simulink model "mars_rover_test_harness_chassis"  (R2025a)
settings: Solver=ode23t  StartTime=0.0  StopTime=30  FixedStep=1e-10  MaxStep=1e-1  RelTol=1e-3  AbsTol=1e-3  EnableMultiTasking=on
undefined symbols (not defined in the file): arm_q0, Control, L1, L2, L3, LS1, LS3, R1, R2, R3, Rover, RS1, RS3, X, Y, Z
libraries: sm_lib x119, nesl_utility x99, fl_lib x85, sdl_lib x20, ee_lib x10, mars_rover_lib x8, simulink x5, slpidlib x3, batteryecm_lib x2
(part 7 of 8)

== system mars_rover_test_harness_chassis/Rover/Chassis/Powertrain/Ideal/Power ==
  i : Inport
  Ambient Temperature : fl_lib/Thermal/Thermal Sources/Temperature Source  temperature=273+25 K
  Battery : batteryecm_lib/Battery  Vnom=14 V  prm_dir=1  R1_dis=2 Ohm  R1_ch=2 Ohm  R1=2e-3 Ohm  prm_AH=2  AH=100 A*hr  V1=11.5 V  AH1=100/2 A*hr  prm_R2=1  R2=2000 Ohm  Tmeas=298.15 K  charge_measurement_port=simscape.enum.battery.enable.yes  prm_dyn=1  Rp1=0.005 Ohm  tau1=30 s  Rp2=0.005 Ohm  tau2=30 s  Rp3=0.005 Ohm  tau3=30 s  Rp4=0.005 Ohm  tau4=30 s  Rp5=0.005 Ohm  tau5=30 s  prm_fade=1  N_fade=100  AH_fade=45 A*hr  R1_fade=2.02 Ohm  R1_ch_fade=2.02 Ohm  V1_fade=10.35 V  prm_age=1  prm_age_OCV=1  OCV_age=0.9  SOC_age=60  Tmeas_age=298.15 K  delta_time_age_vec=[0] d  temperature_age_vec=[273] K  OCV_scaling_age=2.2134e6  OCV_offset_age=1.632e6  temp_exp_age=0.515833569 V  t_exp_age=0.75  Vnom_T2=12 V  R1_T2=2e-2 Ohm  R1_T2_dis=2.2 Ohm  R1_T2_ch=2.2 Ohm  V1_T2=11.4 V  R2_T2=2200 Ohm  Rp1_T2=0.005 Ohm  tau1_T2=30 s  Rp2_T2=0.005 Ohm  tau2_T2=30 s  Rp3_T2=0.005 Ohm  tau3_T2=30 s  Rp4_T2=0.005 Ohm  tau4_T2=30 s  Rp5_T2=0.005 Ohm  tau5_T2=30 s  Tmeas2=273.15 K  thermal_port=simscape.enum.thermaleffects.model  thermal_mass=30000 J/K  i_specify=off  i_priority=None  i=0 A  i_nominal_specify=off  i_nominal_value=1  i_nominal_unit=A  v_specify=off  v_priority=None  v=0 V  v_nominal_specify=off  v_nominal_value=1  v_nominal_unit=V  charge_specify=on  charge_priority=High  charge=100 A*hr  charge_nominal_specify=off  charge_nominal_value=1  charge_nominal_unit=A*hr  num_cycles_specify=off  num_cycles_priority=High  num_cycles=0  num_cycles_nominal_specify=off  num_cycles_nominal_value=1  num_cycles_nominal_unit=1  temperature_specify=on  temperature_priority=High  temperature=288.15 K  temperature_nominal_specify=off  temperature_nominal_value=1  temperature_nominal_unit=K
      settings: InternalSimscapePortConfiguration="{\"Bottom\":[],\"Left\":[{\"id\":\"p\",\"label\":\"+\",\"type\":\"foundation.electrical.electrical\"},{\"id\":\"q\",\"label\":\"q\",\"type\":\"output\"}],\"Right\":[{\"id\":\"n\",\"label\":\"-\",\"type\":\"foundation.electrical.electrical\"},{\"id\":\"H\",\"label\":\"H\",\"type\":\"foundation.thermal.thermal\"}],\"Top\":[]}"
  Controlled Current Source : fl_lib/Electrical/Electrical Sources/Controlled Current Source
  Convective Heat Transfer : fl_lib/Thermal/Thermal Elements/Convective Heat Transfer  thermal_type=foundation.enum.constant_variable.constant  area=1e-4 m^2  heat_tr_coeff=20 W/(m^2 * K)  min_heat_tr_coeff=1e-3 W/(K*m^2)  T_specify=off  T_priority=None  T=0 K  T_nominal_specify=off  T_nominal_value=1  T_nominal_unit=K  Q_specify=off  Q_priority=None  Q=0 W  Q_nominal_specify=off  Q_nominal_value=1  Q_nominal_unit=W
  Electrical Reference : fl_lib/Electrical/Electrical Elements/Electrical Reference
  PS-Simulink Converter : nesl_utility/PS-Simulink Converter  PhysicalDomain=network_engine_domain  SubClassName=ps_output  LeftPortType=input  RightPortType=output  PseudoPeriodic=off  Frequencies=[]  VectorFormat=1-D array  Unit=hr*A  AffineConversion=off
  Sensing Temperature : Subsystem
  Simulink-PS Converter : nesl_utility/Simulink-PS Converter  PhysicalDomain=network_engine_domain  SubClassName=ps_input  LeftPortType=input  RightPortType=output  PseudoPeriodic=off  Frequencies=[]  NoiseDistribution=none  NoiseParameters=[]  Unit=1  AffineConversion=off  FilteringAndDerivatives=provide  SimscapeFilterOrder=1  InputFilterTimeConstant=0.001  UdotUserProvided=0
  Solver Configuration : nesl_utility/Solver Configuration  PhysicalDomain=network_engine_domain  SubClassName=solver  LeftPortType=input  RightPortType=generic  Tones=[]  Harmonics=[]  SimulateNoise=off  Profile=off  UseLocalSampling=off  EnableSwitchedLinearOptims=on  FrequencyDomain=off  UseCCode=off  RelTol=0.001  AbsTol=1e-06  MinStep=1e-09  ToWorkspace=off  RevertToSquareIcSolve=off  NumHomotopyIterations=100  PhasorMode=off  PhasorModeNumHarmonics=1  ConsistencySolver=NEWTON_FTOL  IndexReductionMethod=DerivativeReplacement  DoDC=off  ResidualTolerance=1e-09  ConsistencyTolSource=GLOBAL  ConsistencyAbsTol=0.001  ConsistencyRelTol=0.001  ConsistencyTolFactor=0.001  UseLocalSolver=off  LocalSolverChoice=NE_BACKWARD_EULER_ADVANCER  ResolveIndetEquations=on  FunctionEvalNumThread=1  LocalSolverSampleTime=0.001  DoFixedCost=off  MaxNonlinIter=3  MaxModeIter=2  ComputeImpulses=off  ImpulseIterations=2  LinearAlgebra=auto  LinearAlgebraNumThread=0  EquationFormulation=NE_TIME_EF  DelaysMemoryBudget=1024  AutomaticFiltering=on  FilteringTimeConstant=0.001  PartitionStorageMethod=AS_NEEDED  PartitionMemoryBudget=1024  PartitionMethod=ROBUST  MultibodyUseLocalSolver=off  MultibodyLocalSolverChoice=ODE1  MultibodyLocalSolverSampleTime=0.001
  Out Bus Element4 : Outport  PortName=m  Element=SOC
  Out Bus Element5 : Outport  PortName=m  Element=degC
  wires:
  i/1 -> Simulink-PS Converter/1
  PS-Simulink Converter/1 -> Out Bus Element4/1
  Sensing Temperature/1(T) -> Out Bus Element5/1
  connections:
  Electrical Reference/LConn1 -- Battery/RConn1 -- Controlled Current Source/LConn1 -- Solver Configuration/RConn1
  Battery/LConn1 -- Controlled Current Source/RConn2
  Convective Heat Transfer/RConn1 -- Ambient Temperature/LConn1
  Battery/RConn2 -- Convective Heat Transfer/LConn1 -- Sensing Temperature/LConn1
  PS-Simulink Converter/LConn1 -- Battery/LConn2
  Simulink-PS Converter/RConn1 -- Controlled Current Source/RConn1

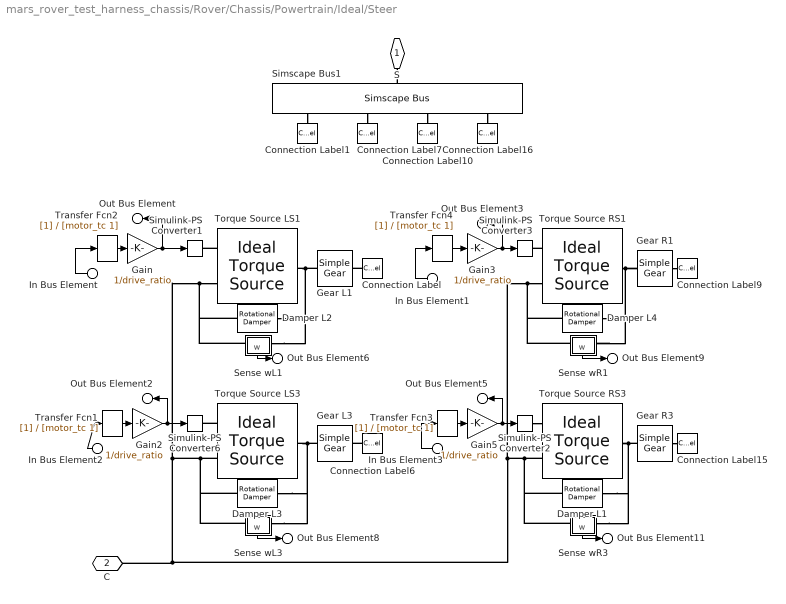
== system mars_rover_test_harness_chassis/Rover/Chassis/Powertrain/Ideal/Steer ==
  In Bus Element : Inport  PortName=Trq  Element=trq.L1
  In Bus Element1 : Inport  PortName=Trq  Element=trq.R1
  In Bus Element2 : Inport  PortName=Trq  Element=trq.L3
  In Bus Element3 : Inport  PortName=Trq  Element=trq.R3
  Connection Label : ConnectionLabel  Label=LS1
  Connection Label1 : ConnectionLabel  Label=LS1
  Connection Label10 : ConnectionLabel  Label=RS1
  Connection Label15 : ConnectionLabel  Label=RS3
  Connection Label16 : ConnectionLabel  Label=RS3
  Connection Label6 : ConnectionLabel  Label=LS3
  Connection Label7 : ConnectionLabel  Label=LS3
  Connection Label9 : ConnectionLabel  Label=RS1
  Damper L{1..4} (4 alike) : fl_lib/Mechanical/Rotational Elements/Rotational Damper  D=motor_d N*m/(rad/s)  w_specify=off  w_priority=None  w=0 rad/s  w_nominal_specify=off  w_nominal_value=1  w_nominal_unit=rad/s  t_specify=off  t_priority=None  t=0 N*m  t_nominal_specify=off  t_nominal_value=1  t_nominal_unit=N*m
  Gain{,2..3,5} (4 alike) : Gain  Gain=1/drive_ratio
  Gear L1 : sdl_lib/Gears/Simple Gear  ratio=drive_ratio  rotation_direction=sdl.enum.shaftOutputDirection.same  friction_model=sdl.enum.gear_efficiencies_load.off  T_noload=0.1 N*m  T_nom=5 N*m  efficiency_nom=0.8  efficiency=drive_efficiency  temperature_TLU=[280, 300, 320] K  load_TLU=[1, 5, 10] N*m  efficiency_TLU=[.95, .9, .85]  efficiency_TLU2=[.85, .8, .75; .95, .9, .85; .85, .8, .7]  w_thr=0.01 rad/s  pwr_thr=0.001 W  enable_backlash=false  hardstop_model=simscape.enum.hardstop.smooth  backlash_distance=1e-3 mm  r_base=0.1 m  transition=1e-4 mm  backlash_stiffness=1e7 N/m  backlash_damping=1e6 N/(m/s)  coeff_rest=0  v_tol=0.001 m/s  f_tol=0 N  mu_visc=[0, 0] N*m/(rad/s)  thermal_mass=50 J/K  temperature_specify=off  temperature_priority=High  temperature=300 K  temperature_nominal_specify=off  temperature_nominal_value=1  temperature_nominal_unit=K  x_backlash_specify=off  x_backlash_priority=None  x_backlash=0 mm  x_backlash_nominal_specify=off  x_backlash_nominal_value=1  x_backlash_nominal_unit=mm  f_hardstop_specify=off  f_hardstop_priority=None  f_hardstop=0 N  f_hardstop_nominal_specify=off  f_hardstop_nominal_value=1  f_hardstop_nominal_unit=N  v_backlash_specify=off  v_backlash_priority=None  v_backlash=0 m/s  v_backlash_nominal_specify=off  v_backlash_nominal_value=1  v_backlash_nominal_unit=m/s
  Gear L3 : sdl_lib/Gears/Simple Gear  ratio=drive_ratio  rotation_direction=sdl.enum.shaftOutputDirection.same  friction_model=sdl.enum.gear_efficiencies_load.off  T_noload=0.1 N*m  T_nom=5 N*m  efficiency_nom=0.8  efficiency=drive_efficiency  temperature_TLU=[280, 300, 320] K  load_TLU=[1, 5, 10] N*m  efficiency_TLU=[.95, .9, .85]  efficiency_TLU2=[.85, .8, .75; .95, .9, .85; .85, .8, .7]  w_thr=0.01 rad/s  pwr_thr=0.001 W  enable_backlash=false  hardstop_model=simscape.enum.hardstop.smooth  backlash_distance=1e-3 mm  r_base=0.1 m  transition=1e-4 mm  backlash_stiffness=1e7 N/m  backlash_damping=1e6 N/(m/s)  coeff_rest=0  v_tol=0.001 m/s  f_tol=0 N  mu_visc=[0, 0] N*m/(rad/s)  thermal_mass=50 J/K  temperature_specify=off  temperature_priority=High  temperature=300 K  temperature_nominal_specify=off  temperature_nominal_value=1  temperature_nominal_unit=K  x_backlash_specify=off  x_backlash_priority=None  x_backlash=0 mm  x_backlash_nominal_specify=off  x_backlash_nominal_value=1  x_backlash_nominal_unit=mm  f_hardstop_specify=off  f_hardstop_priority=None  f_hardstop=0 N  f_hardstop_nominal_specify=off  f_hardstop_nominal_value=1  f_hardstop_nominal_unit=N  v_backlash_specify=off  v_backlash_priority=None  v_backlash=0 m/s  v_backlash_nominal_specify=off  v_backlash_nominal_value=1  v_backlash_nominal_unit=m/s
  Gear R1 : sdl_lib/Gears/Simple Gear  ratio=drive_ratio  rotation_direction=sdl.enum.shaftOutputDirection.same  friction_model=sdl.enum.gear_efficiencies_load.off  T_noload=0.1 N*m  T_nom=5 N*m  efficiency_nom=0.8  efficiency=drive_efficiency  temperature_TLU=[280, 300, 320] K  load_TLU=[1, 5, 10] N*m  efficiency_TLU=[.95, .9, .85]  efficiency_TLU2=[.85, .8, .75; .95, .9, .85; .85, .8, .7]  w_thr=0.01 rad/s  pwr_thr=0.001 W  enable_backlash=false  hardstop_model=simscape.enum.hardstop.smooth  backlash_distance=1e-3 mm  r_base=0.1 m  transition=1e-4 mm  backlash_stiffness=1e7 N/m  backlash_damping=1e6 N/(m/s)  coeff_rest=0  v_tol=0.001 m/s  f_tol=0 N  mu_visc=[0, 0] N*m/(rad/s)  thermal_mass=50 J/K  temperature_specify=off  temperature_priority=High  temperature=300 K  temperature_nominal_specify=off  temperature_nominal_value=1  temperature_nominal_unit=K  x_backlash_specify=off  x_backlash_priority=None  x_backlash=0 mm  x_backlash_nominal_specify=off  x_backlash_nominal_value=1  x_backlash_nominal_unit=mm  f_hardstop_specify=off  f_hardstop_priority=None  f_hardstop=0 N  f_hardstop_nominal_specify=off  f_hardstop_nominal_value=1  f_hardstop_nominal_unit=N  v_backlash_specify=off  v_backlash_priority=None  v_backlash=0 m/s  v_backlash_nominal_specify=off  v_backlash_nominal_value=1  v_backlash_nominal_unit=m/s
  Gear R3 : sdl_lib/Gears/Simple Gear  ratio=drive_ratio  rotation_direction=sdl.enum.shaftOutputDirection.same  friction_model=sdl.enum.gear_efficiencies_load.off  T_noload=0.1 N*m  T_nom=5 N*m  efficiency_nom=0.8  efficiency=drive_efficiency  temperature_TLU=[280, 300, 320] K  load_TLU=[1, 5, 10] N*m  efficiency_TLU=[.95, .9, .85]  efficiency_TLU2=[.85, .8, .75; .95, .9, .85; .85, .8, .7]  w_thr=0.01 rad/s  pwr_thr=0.001 W  enable_backlash=false  hardstop_model=simscape.enum.hardstop.smooth  backlash_distance=1e-3 mm  r_base=0.1 m  transition=1e-4 mm  backlash_stiffness=1e7 N/m  backlash_damping=1e6 N/(m/s)  coeff_rest=0  v_tol=0.001 m/s  f_tol=0 N  mu_visc=[0, 0] N*m/(rad/s)  thermal_mass=50 J/K  temperature_specify=off  temperature_priority=High  temperature=300 K  temperature_nominal_specify=off  temperature_nominal_value=1  temperature_nominal_unit=K  x_backlash_specify=off  x_backlash_priority=None  x_backlash=0 mm  x_backlash_nominal_specify=off  x_backlash_nominal_value=1  x_backlash_nominal_unit=mm  f_hardstop_specify=off  f_hardstop_priority=None  f_hardstop=0 N  f_hardstop_nominal_specify=off  f_hardstop_nominal_value=1  f_hardstop_nominal_unit=N  v_backlash_specify=off  v_backlash_priority=None  v_backlash=0 m/s  v_backlash_nominal_specify=off  v_backlash_nominal_value=1  v_backlash_nominal_unit=m/s
  Sense wL1 : Subsystem
      settings: PortSchema="{\"entries\":[{\"content\":{\"sides\":[{\"content\":{\"connectorIds\":[\"LConn1\"]},\"type\":\"ConnectorPlacement.EquallySpacedRectSide\",\"uuid\":\"592cc1a1-656f-47ce-ad3a-4b4dc1070b5c\"},{\"content\":{\"connectorIds\":[\"RConn1\"],\"side\":\"RIGHT\"},\"type\":\"ConnectorPlacement.EquallySpacedRectSide\",\"uuid\":\"9bca39c3-eeb4-4456-9b97-61ec2f027d42\"},{\"content\":{\"connectorIds\":[],\"side\":\"TOP\"},\"type\":\"ConnectorPlacement.EquallySpacedRectSide\",\"uuid\":\"1e04bf27-fb0c-4be4-96d5-7a7c6152a7df\"},{\"content\":{\"connectorIds\":[\"Out1\"],\"side\":\"BOTTOM\"},\"type\":\"ConnectorPlacement.EquallySpacedRectSide\",\"uuid\":\"fcca2b0e-3afa-4320-884d-439bb49264b6\"}]},\"type\":\"ConnectorPlacement.EquallySpacedConnector\",\"uuid\":\"70eba8cc-e966-48e4-a1ce-5ccb9693dc60\"}],\"packageUris\":[\"http://schema.mathworks.com/mf0/Connector/R2020b\"],\"version\":\"1.0\"}"
      mask Display: disp('w');
  Sense wL3 : Subsystem
      settings: PortSchema="{\"entries\":[{\"content\":{\"sides\":[{\"content\":{\"connectorIds\":[\"LConn1\"]},\"type\":\"ConnectorPlacement.EquallySpacedRectSide\",\"uuid\":\"592cc1a1-656f-47ce-ad3a-4b4dc1070b5c\"},{\"content\":{\"connectorIds\":[\"RConn1\"],\"side\":\"RIGHT\"},\"type\":\"ConnectorPlacement.EquallySpacedRectSide\",\"uuid\":\"9bca39c3-eeb4-4456-9b97-61ec2f027d42\"},{\"content\":{\"connectorIds\":[],\"side\":\"TOP\"},\"type\":\"ConnectorPlacement.EquallySpacedRectSide\",\"uuid\":\"1e04bf27-fb0c-4be4-96d5-7a7c6152a7df\"},{\"content\":{\"connectorIds\":[\"Out1\"],\"side\":\"BOTTOM\"},\"type\":\"ConnectorPlacement.EquallySpacedRectSide\",\"uuid\":\"fcca2b0e-3afa-4320-884d-439bb49264b6\"}]},\"type\":\"ConnectorPlacement.EquallySpacedConnector\",\"uuid\":\"70eba8cc-e966-48e4-a1ce-5ccb9693dc60\"}],\"packageUris\":[\"http://schema.mathworks.com/mf0/Connector/R2020b\"],\"version\":\"1.0\"}"
      mask Display: disp('w');
  Sense wR1 : Subsystem
      settings: PortSchema="{\"entries\":[{\"content\":{\"sides\":[{\"content\":{\"connectorIds\":[\"LConn1\"]},\"type\":\"ConnectorPlacement.EquallySpacedRectSide\",\"uuid\":\"592cc1a1-656f-47ce-ad3a-4b4dc1070b5c\"},{\"content\":{\"connectorIds\":[\"RConn1\"],\"side\":\"RIGHT\"},\"type\":\"ConnectorPlacement.EquallySpacedRectSide\",\"uuid\":\"9bca39c3-eeb4-4456-9b97-61ec2f027d42\"},{\"content\":{\"connectorIds\":[],\"side\":\"TOP\"},\"type\":\"ConnectorPlacement.EquallySpacedRectSide\",\"uuid\":\"1e04bf27-fb0c-4be4-96d5-7a7c6152a7df\"},{\"content\":{\"connectorIds\":[\"Out1\"],\"side\":\"BOTTOM\"},\"type\":\"ConnectorPlacement.EquallySpacedRectSide\",\"uuid\":\"fcca2b0e-3afa-4320-884d-439bb49264b6\"}]},\"type\":\"ConnectorPlacement.EquallySpacedConnector\",\"uuid\":\"70eba8cc-e966-48e4-a1ce-5ccb9693dc60\"}],\"packageUris\":[\"http://schema.mathworks.com/mf0/Connector/R2020b\"],\"version\":\"1.0\"}"
      mask Display: disp('w');
  Sense wR3 : Subsystem
      settings: PortSchema="{\"entries\":[{\"content\":{\"sides\":[{\"content\":{\"connectorIds\":[\"LConn1\"]},\"type\":\"ConnectorPlacement.EquallySpacedRectSide\",\"uuid\":\"592cc1a1-656f-47ce-ad3a-4b4dc1070b5c\"},{\"content\":{\"connectorIds\":[\"RConn1\"],\"side\":\"RIGHT\"},\"type\":\"ConnectorPlacement.EquallySpacedRectSide\",\"uuid\":\"9bca39c3-eeb4-4456-9b97-61ec2f027d42\"},{\"content\":{\"connectorIds\":[],\"side\":\"TOP\"},\"type\":\"ConnectorPlacement.EquallySpacedRectSide\",\"uuid\":\"1e04bf27-fb0c-4be4-96d5-7a7c6152a7df\"},{\"content\":{\"connectorIds\":[\"Out1\"],\"side\":\"BOTTOM\"},\"type\":\"ConnectorPlacement.EquallySpacedRectSide\",\"uuid\":\"fcca2b0e-3afa-4320-884d-439bb49264b6\"}]},\"type\":\"ConnectorPlacement.EquallySpacedConnector\",\"uuid\":\"70eba8cc-e966-48e4-a1ce-5ccb9693dc60\"}],\"packageUris\":[\"http://schema.mathworks.com/mf0/Connector/R2020b\"],\"version\":\"1.0\"}"
      mask Display: disp('w');
  Simscape Bus1 : SimscapeBus  HierarchyStrings=LS1;LS3;RS1;RS3
  Simulink-PS Converter{1..3,6} (4 alike) : nesl_utility/Simulink-PS Converter  PhysicalDomain=network_engine_domain  SubClassName=ps_input  LeftPortType=input  RightPortType=output  PseudoPeriodic=off  Frequencies=[]  NoiseDistribution=none  NoiseParameters=[]  Unit=1  AffineConversion=off  FilteringAndDerivatives=zero  SimscapeFilterOrder=2  InputFilterTimeConstant=0.001  UdotUserProvided=0
  Torque Source LS1 : fl_lib/Mechanical/Mechanical Sources/Ideal Torque Source
  Torque Source LS3 : fl_lib/Mechanical/Mechanical Sources/Ideal Torque Source
  Torque Source RS1 : fl_lib/Mechanical/Mechanical Sources/Ideal Torque Source
  Torque Source RS3 : fl_lib/Mechanical/Mechanical Sources/Ideal Torque Source
  Transfer Fcn{1..4} (4 alike) : TransferFcn  Denominator=[motor_tc 1]
  S : PMIOPort  Side=Right
  C : PMIOPort  Port=2  Side=Left
  Out Bus Element : Outport  PortName=m  Element=trq.L1
  Out Bus Element2 : Outport  PortName=m  Element=trq.L3
  Out Bus Element3 : Outport  PortName=m  Element=trq.R1
  Out Bus Element5 : Outport  PortName=m  Element=trq.R3
  Out Bus Element6 : Outport  PortName=m  Element=w.L1
  Out Bus Element8 : Outport  PortName=m  Element=w.L3
  Out Bus Element9 : Outport  PortName=m  Element=w.R1
  Out Bus Element11 : Outport  PortName=m  Element=w.R3
  wires:
  In Bus Element/1 -> Transfer Fcn2/1
  In Bus Element1/1 -> Transfer Fcn4/1
  In Bus Element2/1 -> Transfer Fcn1/1
  In Bus Element3/1 -> Transfer Fcn3/1
  Gain5/1 -> Out Bus Element5/1, Simulink-PS Converter2/1
  Sense wL3/1(w) -> Out Bus Element8/1
  Gain2/1 -> Out Bus Element2/1, Simulink-PS Converter6/1
  Sense wL1/1(w) -> Out Bus Element6/1
  Gain/1 -> Out Bus Element/1, Simulink-PS Converter1/1
  Sense wR3/1(w) -> Out Bus Element11/1
  Gain3/1 -> Out Bus Element3/1, Simulink-PS Converter3/1
  Sense wR1/1(w) -> Out Bus Element9/1
  Transfer Fcn2/1 -> Gain/1
  Transfer Fcn1/1 -> Gain2/1
  Transfer Fcn3/1 -> Gain5/1
  Transfer Fcn4/1 -> Gain3/1
  connections:
  Gear R3/LConn1 -- Damper L1/LConn1 -- Sense wR3/RConn1 -- Torque Source RS3/LConn1
  Torque Source RS1/LConn1 -- Damper L4/LConn1 -- Sense wR1/RConn1 -- Gear R1/LConn1
  Torque Source RS3/RConn2 -- Damper L1/RConn1 -- Sense wR3/LConn1 -- Damper L4/RConn1 -- Sense wR1/LConn1 -- Torque Source RS1/RConn2 -- Damper L3/RConn1 -- Sense wL3/LConn1 -- Torque Source LS3/RConn2 -- Damper L2/RConn1 -- Sense wL1/LConn1 -- Torque Source LS1/RConn2 -- C/RConn1
  Torque Source LS1/RConn1 -- Simulink-PS Converter1/RConn1
  Gear L1/LConn1 -- Damper L2/LConn1 -- Sense wL1/RConn1 -- Torque Source LS1/LConn1
  Torque Source LS3/RConn1 -- Simulink-PS Converter6/RConn1
  Gear L3/LConn1 -- Damper L3/LConn1 -- Sense wL3/RConn1 -- Torque Source LS3/LConn1
  Simulink-PS Converter2/RConn1 -- Torque Source RS3/RConn1
  Simscape Bus1/LConn1 -- Connection Label1/LConn1
  Simscape Bus1/LConn3 -- Connection Label10/LConn1
  Simscape Bus1/LConn2 -- Connection Label7/LConn1
  Torque Source RS1/RConn1 -- Simulink-PS Converter3/RConn1
  Simscape Bus1/LConn4 -- Connection Label16/LConn1
  Simscape Bus1/RConn1 -- S/RConn1
  Connection Label/LConn1 -- Gear L1/RConn1
  Gear R1/RConn1 -- Connection Label9/LConn1
  Gear R3/RConn1 -- Connection Label15/LConn1
  Connection Label6/LConn1 -- Gear L3/RConn1

== system mars_rover_test_harness_chassis/Rover/Chassis/Roll and Steer/Drive/Camera Frame L1 ==
  Reference Cam Whl : sm_lib/Frames and Transforms/Reference Frame
  Transform Cam Whl : sm_lib/Frames and Transforms/Rigid Transform  RotationMethod=None  FollAlignAxisA=+X  BaseAlignAxisA=+Y  FollAlignAxisB=+Y  BaseAlignAxisB=+Z  RotationStandardAxis=+Z  RotationAngle=0.0  RotationAngleUnits=deg  RotationArbitraryAxis=[0 0 1]  RotationSequenceAxes=FollowerAxes  RotationSequence=XYX  RotationSequenceAngles=[0 0 0]  RotationSequenceAnglesUnits=deg  RotationMatrix=[1 0 0; 0 1 0; 0 0 1]  Quaternion=[1 0 0 0]  TranslationMethod=Cartesian  TranslationCartesianOffset=[0 0 1]  TranslationCartesianOffsetUnits=m  TranslationStandardAxis=+Z  TranslationStandardOffset=0  TranslationStandardOffsetUnits=m  TranslationROffset=0  TranslationROffsetUnits=m  TranslationThetaOffset=0  TranslationThetaOffsetUnits=deg  TranslationZOffset=0  TranslationZOffsetUnits=m
  B : PMIOPort  Side=Left
  connections:
  Transform Cam Whl/LConn1 -- B/RConn1
  Transform Cam Whl/RConn1 -- Reference Cam Whl/RConn1

== system mars_rover_test_harness_chassis/Rover/Chassis/Roll and Steer/Drive/Camera Frame L2 ==
  Reference Cam Whl : sm_lib/Frames and Transforms/Reference Frame
  Transform Cam Whl : sm_lib/Frames and Transforms/Rigid Transform  RotationMethod=None  FollAlignAxisA=+X  BaseAlignAxisA=+Y  FollAlignAxisB=+Y  BaseAlignAxisB=+Z  RotationStandardAxis=+Z  RotationAngle=0.0  RotationAngleUnits=deg  RotationArbitraryAxis=[0 0 1]  RotationSequenceAxes=FollowerAxes  RotationSequence=XYX  RotationSequenceAngles=[0 0 0]  RotationSequenceAnglesUnits=deg  RotationMatrix=[1 0 0; 0 1 0; 0 0 1]  Quaternion=[1 0 0 0]  TranslationMethod=Cartesian  TranslationCartesianOffset=[0 0 1]  TranslationCartesianOffsetUnits=m  TranslationStandardAxis=+Z  TranslationStandardOffset=0  TranslationStandardOffsetUnits=m  TranslationROffset=0  TranslationROffsetUnits=m  TranslationThetaOffset=0  TranslationThetaOffsetUnits=deg  TranslationZOffset=0  TranslationZOffsetUnits=m
  B : PMIOPort  Side=Left
  connections:
  Transform Cam Whl/RConn1 -- Reference Cam Whl/RConn1
  Transform Cam Whl/LConn1 -- B/RConn1

== system mars_rover_test_harness_chassis/Rover/Chassis/Roll and Steer/Drive/Camera Frame L3 ==
  Reference Cam Whl : sm_lib/Frames and Transforms/Reference Frame
  Transform Cam Whl : sm_lib/Frames and Transforms/Rigid Transform  RotationMethod=None  FollAlignAxisA=+X  BaseAlignAxisA=+Y  FollAlignAxisB=+Y  BaseAlignAxisB=+Z  RotationStandardAxis=+Z  RotationAngle=0.0  RotationAngleUnits=deg  RotationArbitraryAxis=[0 0 1]  RotationSequenceAxes=FollowerAxes  RotationSequence=XYX  RotationSequenceAngles=[0 0 0]  RotationSequenceAnglesUnits=deg  RotationMatrix=[1 0 0; 0 1 0; 0 0 1]  Quaternion=[1 0 0 0]  TranslationMethod=Cartesian  TranslationCartesianOffset=[0 0 1]  TranslationCartesianOffsetUnits=m  TranslationStandardAxis=+Z  TranslationStandardOffset=0  TranslationStandardOffsetUnits=m  TranslationROffset=0  TranslationROffsetUnits=m  TranslationThetaOffset=0  TranslationThetaOffsetUnits=deg  TranslationZOffset=0  TranslationZOffsetUnits=m
  B : PMIOPort  Side=Left
  connections:
  Transform Cam Whl/LConn1 -- B/RConn1
  Transform Cam Whl/RConn1 -- Reference Cam Whl/RConn1

== system mars_rover_test_harness_chassis/Rover/Chassis/Roll and Steer/Drive/Camera Frame R1 ==
  Reference Cam Whl : sm_lib/Frames and Transforms/Reference Frame
  Transform Cam Whl : sm_lib/Frames and Transforms/Rigid Transform  RotationMethod=None  FollAlignAxisA=+X  BaseAlignAxisA=+Y  FollAlignAxisB=+Y  BaseAlignAxisB=+Z  RotationStandardAxis=+Z  RotationAngle=0.0  RotationAngleUnits=deg  RotationArbitraryAxis=[0 0 1]  RotationSequenceAxes=FollowerAxes  RotationSequence=XYX  RotationSequenceAngles=[0 0 0]  RotationSequenceAnglesUnits=deg  RotationMatrix=[1 0 0; 0 1 0; 0 0 1]  Quaternion=[1 0 0 0]  TranslationMethod=Cartesian  TranslationCartesianOffset=[0 0 -1]  TranslationCartesianOffsetUnits=m  TranslationStandardAxis=+Z  TranslationStandardOffset=0  TranslationStandardOffsetUnits=m  TranslationROffset=0  TranslationROffsetUnits=m  TranslationThetaOffset=0  TranslationThetaOffsetUnits=deg  TranslationZOffset=0  TranslationZOffsetUnits=m
  B : PMIOPort  Side=Left
  connections:
  Transform Cam Whl/RConn1 -- Reference Cam Whl/RConn1
  Transform Cam Whl/LConn1 -- B/RConn1

== system mars_rover_test_harness_chassis/Rover/Chassis/Roll and Steer/Drive/Camera Frame R2 ==
  Reference Cam Whl : sm_lib/Frames and Transforms/Reference Frame
  Transform Cam Whl : sm_lib/Frames and Transforms/Rigid Transform  RotationMethod=None  FollAlignAxisA=+X  BaseAlignAxisA=+Y  FollAlignAxisB=+Y  BaseAlignAxisB=+Z  RotationStandardAxis=+Z  RotationAngle=0.0  RotationAngleUnits=deg  RotationArbitraryAxis=[0 0 1]  RotationSequenceAxes=FollowerAxes  RotationSequence=XYX  RotationSequenceAngles=[0 0 0]  RotationSequenceAnglesUnits=deg  RotationMatrix=[1 0 0; 0 1 0; 0 0 1]  Quaternion=[1 0 0 0]  TranslationMethod=Cartesian  TranslationCartesianOffset=[0 0 -1]  TranslationCartesianOffsetUnits=m  TranslationStandardAxis=+Z  TranslationStandardOffset=0  TranslationStandardOffsetUnits=m  TranslationROffset=0  TranslationROffsetUnits=m  TranslationThetaOffset=0  TranslationThetaOffsetUnits=deg  TranslationZOffset=0  TranslationZOffsetUnits=m
  B : PMIOPort  Side=Left
  connections:
  Transform Cam Whl/LConn1 -- B/RConn1
  Transform Cam Whl/RConn1 -- Reference Cam Whl/RConn1

== system mars_rover_test_harness_chassis/Rover/Chassis/Roll and Steer/Drive/Camera Frame R3 ==
  Reference Cam Whl : sm_lib/Frames and Transforms/Reference Frame
  Transform Cam Whl : sm_lib/Frames and Transforms/Rigid Transform  RotationMethod=None  FollAlignAxisA=+X  BaseAlignAxisA=+Y  FollAlignAxisB=+Y  BaseAlignAxisB=+Z  RotationStandardAxis=+Z  RotationAngle=0.0  RotationAngleUnits=deg  RotationArbitraryAxis=[0 0 1]  RotationSequenceAxes=FollowerAxes  RotationSequence=XYX  RotationSequenceAngles=[0 0 0]  RotationSequenceAnglesUnits=deg  RotationMatrix=[1 0 0; 0 1 0; 0 0 1]  Quaternion=[1 0 0 0]  TranslationMethod=Cartesian  TranslationCartesianOffset=[0 0 -1]  TranslationCartesianOffsetUnits=m  TranslationStandardAxis=+Z  TranslationStandardOffset=0  TranslationStandardOffsetUnits=m  TranslationROffset=0  TranslationROffsetUnits=m  TranslationThetaOffset=0  TranslationThetaOffsetUnits=deg  TranslationZOffset=0  TranslationZOffsetUnits=m
  B : PMIOPort  Side=Left
  connections:
  Transform Cam Whl/RConn1 -- Reference Cam Whl/RConn1
  Transform Cam Whl/LConn1 -- B/RConn1

== system mars_rover_test_harness_chassis/Rover/Chassis/Roll and Steer/Steer/Steering Bracket L1 ==
  File Solid5 : sm_lib/Body Elements/File Solid  ExtGeomFileName=rover_chassis_steering_bracket.stl  UnitType=Custom  ExtGeomFileUnits=cm  StepReaderType=HEX  ExportConvexHullGeometry=off  InertiaType=CalculateFromGeometry  BasedOnType=Density  Density=1000  DensityUnits=kg/m^3  Mass=0  MassUnits=kg  CenterOfMass=[0 0 0]  CenterOfMassUnits=m  MomentsOfInertia=[1 1 1]*0  MomentsOfInertiaUnits=kg*m^2  ProductsOfInertia=[0 0 0]  ProductsOfInertiaUnits=kg*m^2  GraphicType=FromGeometry  MarkerShape=Sphere  MarkerSize=10  GraphicVisPropType=AdvancedVisualProperties  GraphicDiffuseColor=[0.2 0.2 0.2]  GraphicOpacity=1.0  GraphicSpecularColor=[1 1 1 1.0]  GraphicAmbientColor=[0.15 0.15 0.15 1.0]  GraphicEmissiveColor=[0.0 0.0 0.0 1.0]  GraphicShininess=90  DoExposeReferenceFrame=on  SerializedFrames=<Frames/>
  Reference Frame : sm_lib/Frames and Transforms/Reference Frame
  Rigid Transform : sm_lib/Frames and Transforms/Rigid Transform  RotationMethod=RotationMatrix  FollAlignAxisA=+X  BaseAlignAxisA=+Y  FollAlignAxisB=+Y  BaseAlignAxisB=+Z  RotationStandardAxis=+Z  RotationAngle=0.0  RotationAngleUnits=deg  RotationArbitraryAxis=[0 0 1]  RotationSequenceAxes=FollowerAxes  RotationSequence=XYX  RotationSequenceAngles=[0 0 0]  RotationSequenceAnglesUnits=deg  RotationMatrix=Rover.SteerBracket.SRJ_R  Quaternion=[1 0 0 0]  TranslationMethod=Cartesian  TranslationCartesianOffset=Rover.SteerBracket.SRJ_T  TranslationCartesianOffsetUnits=m  TranslationStandardAxis=+Z  TranslationStandardOffset=0  TranslationStandardOffsetUnits=m  TranslationROffset=0  TranslationROffsetUnits=m  TranslationThetaOffset=0  TranslationThetaOffsetUnits=deg  TranslationZOffset=0  TranslationZOffsetUnits=m
  Rigid Transform1 : sm_lib/Frames and Transforms/Rigid Transform  RotationMethod=RotationMatrix  FollAlignAxisA=+X  BaseAlignAxisA=+Y  FollAlignAxisB=+Y  BaseAlignAxisB=+Z  RotationStandardAxis=+Z  RotationAngle=0.0  RotationAngleUnits=deg  RotationArbitraryAxis=[0 0 1]  RotationSequenceAxes=FollowerAxes  RotationSequence=XYX  RotationSequenceAngles=[0 0 0]  RotationSequenceAnglesUnits=deg  RotationMatrix=Rover.SteerBracket.WRJ_R  Quaternion=[1 0 0 0]  TranslationMethod=Cartesian  TranslationCartesianOffset=Rover.SteerBracket.WRJ_T  TranslationCartesianOffsetUnits=m  TranslationStandardAxis=+Z  TranslationStandardOffset=0  TranslationStandardOffsetUnits=m  TranslationROffset=0  TranslationROffsetUnits=m  TranslationThetaOffset=0  TranslationThetaOffsetUnits=deg  TranslationZOffset=0  TranslationZOffsetUnits=m
  B : PMIOPort  Side=Left
  F : PMIOPort  Port=2  Side=Right
  connections:
  Rigid Transform/LConn1 -- Rigid Transform1/LConn1 -- Reference Frame/RConn1 -- File Solid5/RConn1
  F/RConn1 -- Rigid Transform1/RConn1
  Rigid Transform/RConn1 -- B/RConn1

== system mars_rover_test_harness_chassis/Rover/Chassis/Roll and Steer/Steer/Steering Bracket L3 ==
  File Solid5 : sm_lib/Body Elements/File Solid  ExtGeomFileName=rover_chassis_steering_bracket.stl  UnitType=Custom  ExtGeomFileUnits=cm  StepReaderType=HEX  ExportConvexHullGeometry=off  InertiaType=CalculateFromGeometry  BasedOnType=Density  Density=1000  DensityUnits=kg/m^3  Mass=0  MassUnits=kg  CenterOfMass=[0 0 0]  CenterOfMassUnits=m  MomentsOfInertia=[1 1 1]*0  MomentsOfInertiaUnits=kg*m^2  ProductsOfInertia=[0 0 0]  ProductsOfInertiaUnits=kg*m^2  GraphicType=FromGeometry  MarkerShape=Sphere  MarkerSize=10  GraphicVisPropType=AdvancedVisualProperties  GraphicDiffuseColor=[0.2 0.2 0.2]  GraphicOpacity=1.0  GraphicSpecularColor=[1 1 1 1.0]  GraphicAmbientColor=[0.15 0.15 0.15 1.0]  GraphicEmissiveColor=[0.0 0.0 0.0 1.0]  GraphicShininess=90  DoExposeReferenceFrame=on  SerializedFrames=<Frames/>
  Reference Frame : sm_lib/Frames and Transforms/Reference Frame
  Rigid Transform : sm_lib/Frames and Transforms/Rigid Transform  RotationMethod=RotationMatrix  FollAlignAxisA=+X  BaseAlignAxisA=+Y  FollAlignAxisB=+Y  BaseAlignAxisB=+Z  RotationStandardAxis=+Z  RotationAngle=0.0  RotationAngleUnits=deg  RotationArbitraryAxis=[0 0 1]  RotationSequenceAxes=FollowerAxes  RotationSequence=XYX  RotationSequenceAngles=[0 0 0]  RotationSequenceAnglesUnits=deg  RotationMatrix=Rover.SteerBracket.SRJ_R  Quaternion=[1 0 0 0]  TranslationMethod=Cartesian  TranslationCartesianOffset=Rover.SteerBracket.SRJ_T  TranslationCartesianOffsetUnits=m  TranslationStandardAxis=+Z  TranslationStandardOffset=0  TranslationStandardOffsetUnits=m  TranslationROffset=0  TranslationROffsetUnits=m  TranslationThetaOffset=0  TranslationThetaOffsetUnits=deg  TranslationZOffset=0  TranslationZOffsetUnits=m
  Rigid Transform1 : sm_lib/Frames and Transforms/Rigid Transform  RotationMethod=RotationMatrix  FollAlignAxisA=+X  BaseAlignAxisA=+Y  FollAlignAxisB=+Y  BaseAlignAxisB=+Z  RotationStandardAxis=+Z  RotationAngle=0.0  RotationAngleUnits=deg  RotationArbitraryAxis=[0 0 1]  RotationSequenceAxes=FollowerAxes  RotationSequence=XYX  RotationSequenceAngles=[0 0 0]  RotationSequenceAnglesUnits=deg  RotationMatrix=Rover.SteerBracket.WRJ_R  Quaternion=[1 0 0 0]  TranslationMethod=Cartesian  TranslationCartesianOffset=Rover.SteerBracket.WRJ_T  TranslationCartesianOffsetUnits=m  TranslationStandardAxis=+Z  TranslationStandardOffset=0  TranslationStandardOffsetUnits=m  TranslationROffset=0  TranslationROffsetUnits=m  TranslationThetaOffset=0  TranslationThetaOffsetUnits=deg  TranslationZOffset=0  TranslationZOffsetUnits=m
  B : PMIOPort  Side=Left
  F : PMIOPort  Port=2  Side=Right
  connections:
  File Solid5/RConn1 -- Reference Frame/RConn1 -- Rigid Transform/LConn1 -- Rigid Transform1/LConn1
  F/RConn1 -- Rigid Transform1/RConn1
  Rigid Transform/RConn1 -- B/RConn1

== system mars_rover_test_harness_chassis/Rover/Chassis/Roll and Steer/Steer/Steering Bracket R1 ==
  File Solid5 : sm_lib/Body Elements/File Solid  ExtGeomFileName=rover_chassis_steering_bracket.stl  UnitType=Custom  ExtGeomFileUnits=cm  StepReaderType=HEX  ExportConvexHullGeometry=off  InertiaType=CalculateFromGeometry  BasedOnType=Density  Density=1000  DensityUnits=kg/m^3  Mass=0  MassUnits=kg  CenterOfMass=[0 0 0]  CenterOfMassUnits=m  MomentsOfInertia=[1 1 1]*0  MomentsOfInertiaUnits=kg*m^2  ProductsOfInertia=[0 0 0]  ProductsOfInertiaUnits=kg*m^2  GraphicType=FromGeometry  MarkerShape=Sphere  MarkerSize=10  GraphicVisPropType=AdvancedVisualProperties  GraphicDiffuseColor=[0.2 0.2 0.2]  GraphicOpacity=1.0  GraphicSpecularColor=[1 1 1 1.0]  GraphicAmbientColor=[0.15 0.15 0.15 1.0]  GraphicEmissiveColor=[0.0 0.0 0.0 1.0]  GraphicShininess=90  DoExposeReferenceFrame=on  SerializedFrames=<Frames/>
  Reference Frame : sm_lib/Frames and Transforms/Reference Frame
  Rigid Transform : sm_lib/Frames and Transforms/Rigid Transform  RotationMethod=RotationMatrix  FollAlignAxisA=+X  BaseAlignAxisA=+Y  FollAlignAxisB=+Y  BaseAlignAxisB=+Z  RotationStandardAxis=+Z  RotationAngle=0.0  RotationAngleUnits=deg  RotationArbitraryAxis=[0 0 1]  RotationSequenceAxes=FollowerAxes  RotationSequence=XYX  RotationSequenceAngles=[0 0 0]  RotationSequenceAnglesUnits=deg  RotationMatrix=Rover.SteerBracket.SRJ_R  Quaternion=[1 0 0 0]  TranslationMethod=Cartesian  TranslationCartesianOffset=Rover.SteerBracket.SRJ_T  TranslationCartesianOffsetUnits=m  TranslationStandardAxis=+Z  TranslationStandardOffset=0  TranslationStandardOffsetUnits=m  TranslationROffset=0  TranslationROffsetUnits=m  TranslationThetaOffset=0  TranslationThetaOffsetUnits=deg  TranslationZOffset=0  TranslationZOffsetUnits=m
  Rigid Transform1 : sm_lib/Frames and Transforms/Rigid Transform  RotationMethod=RotationMatrix  FollAlignAxisA=+X  BaseAlignAxisA=+Y  FollAlignAxisB=+Y  BaseAlignAxisB=+Z  RotationStandardAxis=+Z  RotationAngle=0.0  RotationAngleUnits=deg  RotationArbitraryAxis=[0 0 1]  RotationSequenceAxes=FollowerAxes  RotationSequence=XYX  RotationSequenceAngles=[0 0 0]  RotationSequenceAnglesUnits=deg  RotationMatrix=Rover.SteerBracket.WRJ_R  Quaternion=[1 0 0 0]  TranslationMethod=Cartesian  TranslationCartesianOffset=Rover.SteerBracket.WRJ_T  TranslationCartesianOffsetUnits=m  TranslationStandardAxis=+Z  TranslationStandardOffset=0  TranslationStandardOffsetUnits=m  TranslationROffset=0  TranslationROffsetUnits=m  TranslationThetaOffset=0  TranslationThetaOffsetUnits=deg  TranslationZOffset=0  TranslationZOffsetUnits=m
  Transform Right Side : sm_lib/Frames and Transforms/Rigid Transform  RotationMethod=StandardAxis  FollAlignAxisA=+X  BaseAlignAxisA=+Y  FollAlignAxisB=+Y  BaseAlignAxisB=+Z  RotationStandardAxis=+Y  RotationAngle=180  RotationAngleUnits=deg  RotationArbitraryAxis=[0 0 1]  RotationSequenceAxes=FollowerAxes  RotationSequence=XYX  RotationSequenceAngles=[0 0 0]  RotationSequenceAnglesUnits=deg  RotationMatrix=[1 0 0; 0 1 0; 0 0 1]  Quaternion=[1 0 0 0]  TranslationMethod=None  TranslationCartesianOffset=[0 0 0]  TranslationCartesianOffsetUnits=m  TranslationStandardAxis=+Z  TranslationStandardOffset=0  TranslationStandardOffsetUnits=m  TranslationROffset=0  TranslationROffsetUnits=m  TranslationThetaOffset=0  TranslationThetaOffsetUnits=deg  TranslationZOffset=0  TranslationZOffsetUnits=m
  B : PMIOPort  Side=Right
  F : PMIOPort  Port=2  Side=Left
  connections:
  Rigid Transform/LConn1 -- Rigid Transform1/LConn1 -- Reference Frame/RConn1 -- File Solid5/RConn1
  Transform Right Side/RConn1 -- Rigid Transform1/RConn1
  Rigid Transform/RConn1 -- B/RConn1
  Transform Right Side/LConn1 -- F/RConn1

== system mars_rover_test_harness_chassis/Rover/Chassis/Roll and Steer/Steer/Steering Bracket R3 ==
  File Solid5 : sm_lib/Body Elements/File Solid  ExtGeomFileName=rover_chassis_steering_bracket.stl  UnitType=Custom  ExtGeomFileUnits=cm  StepReaderType=HEX  ExportConvexHullGeometry=off  InertiaType=CalculateFromGeometry  BasedOnType=Density  Density=1000  DensityUnits=kg/m^3  Mass=0  MassUnits=kg  CenterOfMass=[0 0 0]  CenterOfMassUnits=m  MomentsOfInertia=[1 1 1]*0  MomentsOfInertiaUnits=kg*m^2  ProductsOfInertia=[0 0 0]  ProductsOfInertiaUnits=kg*m^2  GraphicType=FromGeometry  MarkerShape=Sphere  MarkerSize=10  GraphicVisPropType=AdvancedVisualProperties  GraphicDiffuseColor=[0.2 0.2 0.2]  GraphicOpacity=1.0  GraphicSpecularColor=[1 1 1 1.0]  GraphicAmbientColor=[0.15 0.15 0.15 1.0]  GraphicEmissiveColor=[0.0 0.0 0.0 1.0]  GraphicShininess=90  DoExposeReferenceFrame=on  SerializedFrames=<Frames/>
  Reference Frame : sm_lib/Frames and Transforms/Reference Frame
  Rigid Transform : sm_lib/Frames and Transforms/Rigid Transform  RotationMethod=RotationMatrix  FollAlignAxisA=+X  BaseAlignAxisA=+Y  FollAlignAxisB=+Y  BaseAlignAxisB=+Z  RotationStandardAxis=+Z  RotationAngle=0.0  RotationAngleUnits=deg  RotationArbitraryAxis=[0 0 1]  RotationSequenceAxes=FollowerAxes  RotationSequence=XYX  RotationSequenceAngles=[0 0 0]  RotationSequenceAnglesUnits=deg  RotationMatrix=Rover.SteerBracket.SRJ_R  Quaternion=[1 0 0 0]  TranslationMethod=Cartesian  TranslationCartesianOffset=Rover.SteerBracket.SRJ_T  TranslationCartesianOffsetUnits=m  TranslationStandardAxis=+Z  TranslationStandardOffset=0  TranslationStandardOffsetUnits=m  TranslationROffset=0  TranslationROffsetUnits=m  TranslationThetaOffset=0  TranslationThetaOffsetUnits=deg  TranslationZOffset=0  TranslationZOffsetUnits=m
  Rigid Transform1 : sm_lib/Frames and Transforms/Rigid Transform  RotationMethod=RotationMatrix  FollAlignAxisA=+X  BaseAlignAxisA=+Y  FollAlignAxisB=+Y  BaseAlignAxisB=+Z  RotationStandardAxis=+Z  RotationAngle=0.0  RotationAngleUnits=deg  RotationArbitraryAxis=[0 0 1]  RotationSequenceAxes=FollowerAxes  RotationSequence=XYX  RotationSequenceAngles=[0 0 0]  RotationSequenceAnglesUnits=deg  RotationMatrix=Rover.SteerBracket.WRJ_R  Quaternion=[1 0 0 0]  TranslationMethod=Cartesian  TranslationCartesianOffset=Rover.SteerBracket.WRJ_T  TranslationCartesianOffsetUnits=m  TranslationStandardAxis=+Z  TranslationStandardOffset=0  TranslationStandardOffsetUnits=m  TranslationROffset=0  TranslationROffsetUnits=m  TranslationThetaOffset=0  TranslationThetaOffsetUnits=deg  TranslationZOffset=0  TranslationZOffsetUnits=m
  Transform Right Side : sm_lib/Frames and Transforms/Rigid Transform  RotationMethod=StandardAxis  FollAlignAxisA=+X  BaseAlignAxisA=+Y  FollAlignAxisB=+Y  BaseAlignAxisB=+Z  RotationStandardAxis=+Y  RotationAngle=180  RotationAngleUnits=deg  RotationArbitraryAxis=[0 0 1]  RotationSequenceAxes=FollowerAxes  RotationSequence=XYX  RotationSequenceAngles=[0 0 0]  RotationSequenceAnglesUnits=deg  RotationMatrix=[1 0 0; 0 1 0; 0 0 1]  Quaternion=[1 0 0 0]  TranslationMethod=None  TranslationCartesianOffset=[0 0 0]  TranslationCartesianOffsetUnits=m  TranslationStandardAxis=+Z  TranslationStandardOffset=0  TranslationStandardOffsetUnits=m  TranslationROffset=0  TranslationROffsetUnits=m  TranslationThetaOffset=0  TranslationThetaOffsetUnits=deg  TranslationZOffset=0  TranslationZOffsetUnits=m
  B : PMIOPort  Side=Right
  F : PMIOPort  Port=2  Side=Left
  connections:
  Rigid Transform/RConn1 -- B/RConn1
  Transform Right Side/RConn1 -- Rigid Transform1/RConn1
  File Solid5/RConn1 -- Reference Frame/RConn1 -- Rigid Transform1/LConn1 -- Rigid Transform/LConn1
  Transform Right Side/LConn1 -- F/RConn1

== system mars_rover_test_harness_chassis/Rover/Chassis/Powertrain/Electrical/Drive/Sense tL1 ==
  Ideal Torque Sensor : fl_lib/Mechanical/Mechanical Sensors/Ideal Torque Sensor
  PS-Simulink Converter6 : nesl_utility/PS-Simulink Converter  PhysicalDomain=network_engine_domain  SubClassName=ps_output  LeftPortType=input  RightPortType=output  PseudoPeriodic=off  Frequencies=[]  VectorFormat=1-D array  Unit=inherit  AffineConversion=off
  C : PMIOPort  Side=Right
  R : PMIOPort  Port=2  Side=Left
  T : Outport
  wires:
  PS-Simulink Converter6/1 -> T/1
  connections:
  Ideal Torque Sensor/LConn1 -- R/RConn1
  Ideal Torque Sensor/RConn2 -- PS-Simulink Converter6/LConn1
  Ideal Torque Sensor/RConn1 -- C/RConn1

== system mars_rover_test_harness_chassis/Rover/Chassis/Powertrain/Electrical/Drive/Sense tL2 ==
  Ideal Torque Sensor : fl_lib/Mechanical/Mechanical Sensors/Ideal Torque Sensor
  PS-Simulink Converter6 : nesl_utility/PS-Simulink Converter  PhysicalDomain=network_engine_domain  SubClassName=ps_output  LeftPortType=input  RightPortType=output  PseudoPeriodic=off  Frequencies=[]  VectorFormat=1-D array  Unit=inherit  AffineConversion=off
  C : PMIOPort  Side=Right
  R : PMIOPort  Port=2  Side=Left
  T : Outport
  wires:
  PS-Simulink Converter6/1 -> T/1
  connections:
  Ideal Torque Sensor/RConn1 -- C/RConn1
  Ideal Torque Sensor/RConn2 -- PS-Simulink Converter6/LConn1
  Ideal Torque Sensor/LConn1 -- R/RConn1

== system mars_rover_test_harness_chassis/Rover/Chassis/Powertrain/Electrical/Drive/Sense tL3 ==
  Ideal Torque Sensor : fl_lib/Mechanical/Mechanical Sensors/Ideal Torque Sensor
  PS-Simulink Converter6 : nesl_utility/PS-Simulink Converter  PhysicalDomain=network_engine_domain  SubClassName=ps_output  LeftPortType=input  RightPortType=output  PseudoPeriodic=off  Frequencies=[]  VectorFormat=1-D array  Unit=inherit  AffineConversion=off
  R : PMIOPort  Side=Left
  C : PMIOPort  Port=2  Side=Right
  T : Outport
  wires:
  PS-Simulink Converter6/1 -> T/1
  connections:
  Ideal Torque Sensor/LConn1 -- R/RConn1
  Ideal Torque Sensor/RConn2 -- PS-Simulink Converter6/LConn1
  Ideal Torque Sensor/RConn1 -- C/RConn1

== system mars_rover_test_harness_chassis/Rover/Chassis/Powertrain/Electrical/Drive/Sense tR1 ==
  Ideal Torque Sensor : fl_lib/Mechanical/Mechanical Sensors/Ideal Torque Sensor
  PS-Simulink Converter6 : nesl_utility/PS-Simulink Converter  PhysicalDomain=network_engine_domain  SubClassName=ps_output  LeftPortType=input  RightPortType=output  PseudoPeriodic=off  Frequencies=[]  VectorFormat=1-D array  Unit=inherit  AffineConversion=off
  C : PMIOPort  Side=Right
  R : PMIOPort  Port=2  Side=Left
  T : Outport
  wires:
  PS-Simulink Converter6/1 -> T/1
  connections:
  Ideal Torque Sensor/RConn1 -- C/RConn1
  Ideal Torque Sensor/RConn2 -- PS-Simulink Converter6/LConn1
  Ideal Torque Sensor/LConn1 -- R/RConn1

== system mars_rover_test_harness_chassis/Rover/Chassis/Powertrain/Electrical/Drive/Sense tR2 ==
  Ideal Torque Sensor : fl_lib/Mechanical/Mechanical Sensors/Ideal Torque Sensor
  PS-Simulink Converter6 : nesl_utility/PS-Simulink Converter  PhysicalDomain=network_engine_domain  SubClassName=ps_output  LeftPortType=input  RightPortType=output  PseudoPeriodic=off  Frequencies=[]  VectorFormat=1-D array  Unit=inherit  AffineConversion=off
  C : PMIOPort  Side=Right
  R : PMIOPort  Port=2  Side=Left
  T : Outport
  wires:
  PS-Simulink Converter6/1 -> T/1
  connections:
  Ideal Torque Sensor/LConn1 -- R/RConn1
  Ideal Torque Sensor/RConn2 -- PS-Simulink Converter6/LConn1
  Ideal Torque Sensor/RConn1 -- C/RConn1

== system mars_rover_test_harness_chassis/Rover/Chassis/Powertrain/Electrical/Drive/Sense tR3 ==
  Ideal Torque Sensor : fl_lib/Mechanical/Mechanical Sensors/Ideal Torque Sensor
  PS-Simulink Converter6 : nesl_utility/PS-Simulink Converter  PhysicalDomain=network_engine_domain  SubClassName=ps_output  LeftPortType=input  RightPortType=output  PseudoPeriodic=off  Frequencies=[]  VectorFormat=1-D array  Unit=inherit  AffineConversion=off
  C : PMIOPort  Side=Right
  R : PMIOPort  Port=2  Side=Left
  T : Outport
  wires:
  PS-Simulink Converter6/1 -> T/1
  connections:
  Ideal Torque Sensor/RConn1 -- C/RConn1
  Ideal Torque Sensor/RConn2 -- PS-Simulink Converter6/LConn1
  Ideal Torque Sensor/LConn1 -- R/RConn1

== system mars_rover_test_harness_chassis/Rover/Chassis/Powertrain/Electrical/Drive/Sensor iL1 ==
  Current Sensor : fl_lib/Electrical/Electrical Sensors/Current Sensor
  PS-Simulink Converter3 : nesl_utility/PS-Simulink Converter  PhysicalDomain=network_engine_domain  SubClassName=ps_output  LeftPortType=input  RightPortType=output  PseudoPeriodic=off  Frequencies=[]  VectorFormat=1-D array  Unit=inherit  AffineConversion=off
  + : PMIOPort  Side=Left
  - : PMIOPort  Port=2  Side=Right
  i : Outport
  wires:
  PS-Simulink Converter3/1 -> i/1
  connections:
  PS-Simulink Converter3/LConn1 -- Current Sensor/RConn1
  Current Sensor/RConn2 -- -/RConn1
  +/RConn1 -- Current Sensor/LConn1

== system mars_rover_test_harness_chassis/Rover/Chassis/Powertrain/Electrical/Drive/Sensor iL2 ==
  Current Sensor : fl_lib/Electrical/Electrical Sensors/Current Sensor
  PS-Simulink Converter3 : nesl_utility/PS-Simulink Converter  PhysicalDomain=network_engine_domain  SubClassName=ps_output  LeftPortType=input  RightPortType=output  PseudoPeriodic=off  Frequencies=[]  VectorFormat=1-D array  Unit=inherit  AffineConversion=off
  + : PMIOPort  Side=Left
  - : PMIOPort  Port=2  Side=Right
  i : Outport
  wires:
  PS-Simulink Converter3/1 -> i/1
  connections:
  +/RConn1 -- Current Sensor/LConn1
  Current Sensor/RConn2 -- -/RConn1
  PS-Simulink Converter3/LConn1 -- Current Sensor/RConn1

== system mars_rover_test_harness_chassis/Rover/Chassis/Powertrain/Electrical/Drive/Sensor iL3 ==
  Current Sensor : fl_lib/Electrical/Electrical Sensors/Current Sensor
  PS-Simulink Converter3 : nesl_utility/PS-Simulink Converter  PhysicalDomain=network_engine_domain  SubClassName=ps_output  LeftPortType=input  RightPortType=output  PseudoPeriodic=off  Frequencies=[]  VectorFormat=1-D array  Unit=inherit  AffineConversion=off
  + : PMIOPort  Side=Left
  - : PMIOPort  Port=2  Side=Right
  i : Outport
  wires:
  PS-Simulink Converter3/1 -> i/1
  connections:
  +/RConn1 -- Current Sensor/LConn1
  Current Sensor/RConn2 -- -/RConn1
  PS-Simulink Converter3/LConn1 -- Current Sensor/RConn1

== system mars_rover_test_harness_chassis/Rover/Chassis/Powertrain/Electrical/Drive/Sensor iR1 ==
  Current Sensor : fl_lib/Electrical/Electrical Sensors/Current Sensor
  PS-Simulink Converter3 : nesl_utility/PS-Simulink Converter  PhysicalDomain=network_engine_domain  SubClassName=ps_output  LeftPortType=input  RightPortType=output  PseudoPeriodic=off  Frequencies=[]  VectorFormat=1-D array  Unit=inherit  AffineConversion=off
  + : PMIOPort  Side=Left
  - : PMIOPort  Port=2  Side=Right
  i : Outport
  wires:
  PS-Simulink Converter3/1 -> i/1
  connections:
  +/RConn1 -- Current Sensor/LConn1
  Current Sensor/RConn2 -- -/RConn1
  PS-Simulink Converter3/LConn1 -- Current Sensor/RConn1

== system mars_rover_test_harness_chassis/Rover/Chassis/Powertrain/Electrical/Drive/Sensor iR2 ==
  Current Sensor : fl_lib/Electrical/Electrical Sensors/Current Sensor
  PS-Simulink Converter3 : nesl_utility/PS-Simulink Converter  PhysicalDomain=network_engine_domain  SubClassName=ps_output  LeftPortType=input  RightPortType=output  PseudoPeriodic=off  Frequencies=[]  VectorFormat=1-D array  Unit=inherit  AffineConversion=off
  + : PMIOPort  Side=Left
  - : PMIOPort  Port=2  Side=Right
  i : Outport
  wires:
  PS-Simulink Converter3/1 -> i/1
  connections:
  PS-Simulink Converter3/LConn1 -- Current Sensor/RConn1
  Current Sensor/RConn2 -- -/RConn1
  +/RConn1 -- Current Sensor/LConn1

== system mars_rover_test_harness_chassis/Rover/Chassis/Powertrain/Electrical/Drive/Sensor iR3 ==
  Current Sensor : fl_lib/Electrical/Electrical Sensors/Current Sensor
  PS-Simulink Converter3 : nesl_utility/PS-Simulink Converter  PhysicalDomain=network_engine_domain  SubClassName=ps_output  LeftPortType=input  RightPortType=output  PseudoPeriodic=off  Frequencies=[]  VectorFormat=1-D array  Unit=inherit  AffineConversion=off
  + : PMIOPort  Side=Left
  - : PMIOPort  Port=2  Side=Right
  i : Outport
  wires:
  PS-Simulink Converter3/1 -> i/1
  connections:
  PS-Simulink Converter3/LConn1 -- Current Sensor/RConn1
  Current Sensor/RConn2 -- -/RConn1
  +/RConn1 -- Current Sensor/LConn1

== system mars_rover_test_harness_chassis/Rover/Chassis/Powertrain/Electrical/Power/Sensing Temperature ==
  PS-Simulink Converter : nesl_utility/PS-Simulink Converter  PhysicalDomain=network_engine_domain  SubClassName=ps_output  LeftPortType=input  RightPortType=output  PseudoPeriodic=off  Frequencies=[]  VectorFormat=1-D array  Unit=inherit  AffineConversion=off
  Temperature Sensor : fl_lib/Thermal/Thermal Sensors/Temperature Sensor  temperature_measure=foundation.enum.MeasurementReference.difference
  Thermal Reference : fl_lib/Thermal/Thermal Elements/Thermal Reference
  A : PMIOPort  Side=Left
  T : Outport
  wires:
  PS-Simulink Converter/1 -> T/1
  connections:
  Thermal Reference/LConn1 -- Temperature Sensor/RConn1
  Temperature Sensor/RConn2 -- PS-Simulink Converter/LConn1
  A/RConn1 -- Temperature Sensor/LConn1

== system mars_rover_test_harness_chassis/Rover/Chassis/Powertrain/Electrical/Steer/Sense T1 ==
  Ideal Torque Sensor : fl_lib/Mechanical/Mechanical Sensors/Ideal Torque Sensor
  PS-Simulink Converter6 : nesl_utility/PS-Simulink Converter  PhysicalDomain=network_engine_domain  SubClassName=ps_output  LeftPortType=input  RightPortType=output  PseudoPeriodic=off  Frequencies=[]  VectorFormat=1-D array  Unit=inherit  AffineConversion=off
  C : PMIOPort  Side=Right
  R : PMIOPort  Port=2  Side=Left
  T : Outport
  wires:
  PS-Simulink Converter6/1 -> T/1
  connections:
  Ideal Torque Sensor/LConn1 -- R/RConn1
  Ideal Torque Sensor/RConn2 -- PS-Simulink Converter6/LConn1
  Ideal Torque Sensor/RConn1 -- C/RConn1
